simulink model "halfWaveUncontrolledRectifier_RLload"  (R2024b)
settings: Solver=ode23t  StartTime=0.0  StopTime=0.16  MaxStep=1e-4  RelTol=1e-3
libraries: spsVoltageMeasurementLib x3, spsSeriesRLCBranchLib x2, spsACVoltageSourceLib x1, spsDiodeLib x1, spsCurrentMeasurementLib x1, sps_lib x1
settings Model: Creator=farha  LastModifiedBy=farha

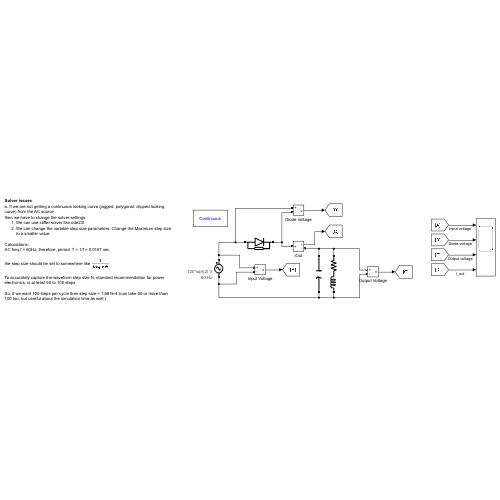
[thumbnail: Simulink's stored preview of the top-level diagram]
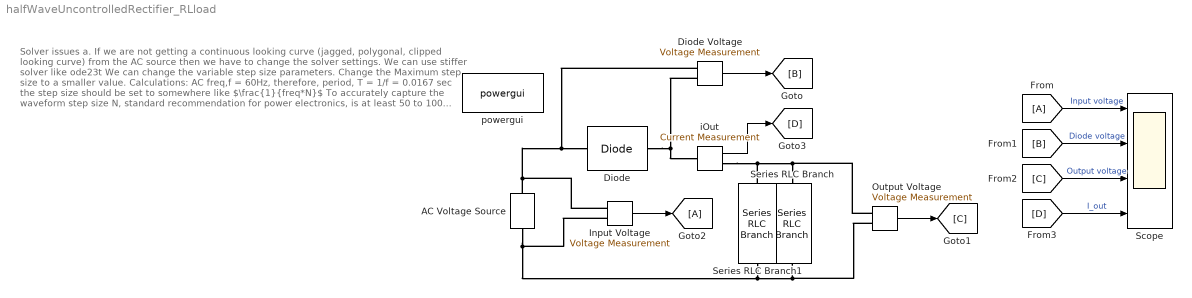
== system halfWaveUncontrolledRectifier_RLload ==
  note: Solver issues
      | a. If we are not getting a continuous looking curve (jagged, polygonal, clipped looking curve) from the AC source
      | then we have to change the solver settings.
      | We can use stiffer solver like ode23t
      | We can change the variable step size parameters. Change the Maximum step size to a smaller value.
      |
      | Calculations:
      | AC freq,f = 60Hz, therefore, period, T = 1/f = 0.0167 sec
      |
      | the step size should be set to somewhere like $\frac{1}{freq*N}$
      |
      | To accurately capture the waveform step size N, standard recommendation for power electronics, is at least 50 to 100 steps
      |
      | So, if we want 100 steps per cycle then step size = 1.667e-4 (can take 50 or more than 100 too, but careful about the simulation time as well.)
  AC Voltage Source : spsACVoltageSourceLib/AC Voltage Source  Amplitude=120*sqrt(2)  Phase=0  Frequency=60  SampleTime=0  Measurements=None  BusType=swing  Pref=10e3  Qref=0  Qmin=-inf  Qmax=+inf
      settings: AttributesFormatString=|
      | %<Amplitude> V
      | %<Frequency> Hz
  Diode : spsDiodeLib/Diode  Ron=0.001  Lon=0  Vf=0.8  IC=0  UseSnubber=0  Rs=500  Cs=250e-9  Measurements=off
  Diode Voltage : spsVoltageMeasurementLib/Voltage Measurement  PhasorSimulation=off  OutputType=Complex  PSBequivalent=0
  From : From
  Goto2 : Goto
  Input Voltage : spsVoltageMeasurementLib/Voltage Measurement  PhasorSimulation=off  OutputType=Complex  PSBequivalent=0
  Output Voltage : spsVoltageMeasurementLib/Voltage Measurement  PhasorSimulation=off  OutputType=Complex  PSBequivalent=0
  Scope : Scope  NumInputPorts=4
  Series RLC Branch : spsSeriesRLCBranchLib/Series RLC Branch  LConnTagsString=__new0  RConnTagsString=__new0  BranchType=RL  Resistance=100  Inductance=0.1  SetiL0=off  InitialCurrent=0  Capacitance=1e-6  Setx0=off  InitialVoltage=0  Measurements=None
  Series RLC Branch1 : spsSeriesRLCBranchLib/Series RLC Branch  LConnTagsString=__new0  RConnTagsString=__new0  BranchType=C  Resistance=5  Inductance=1e-3  SetiL0=off  InitialCurrent=0  Capacitance=220e-6  Setx0=off  InitialVoltage=0  Measurements=None
  iOut : spsCurrentMeasurementLib/Current Measurement  PhasorSimulation=off  OutputType=Complex  PSBequivalent=0
  powergui : sps_lib/powergui  Priority=1  SimulationMode=Continuous  SampleTime=50e-6  frequency=60  Iterations=50  frequencyindice=60  Pbase=100e6  ErrMax=1e-4  UnitsV=kV  UnitsW=MW  buscounter=0  FunctionMessages=off  echomessages=off  EnableUseOfTLC=off  CurrentSourceSwitches=off  DisableSnubberDevices=off  DisableRonSwitches=off  DisableVfSwitches=off  DisplayEquations=off  AutomaticDiscreteSolvers=off  SolverType=Tustin/Backward Euler (TBE)  Interpol=off  ExternalGateDelay=off  methode=off  Ts=100  x0status=blocks  SPID=on  SwTol=0  HookPort=off  NonlinearTolerance=1e-4  nMaxIteration=100  ContinueOnMaxIteration=off  RestoreLinks=warning  ResistiveCurrentMeasurement=off  Frange=[0:2:500]  Ylog=off  Xlog=on  ShowGrid=off  save=off  variable=ZData  structure=0  ZoomFFT=off  StartTime=0.0  cycles=1  DisplayStyle=1  fundamental=60  FreqAxis=off  MaxFrequency=1000  frequencyindicesteady=1  RmsSteady=1  display=off
  wires:
  Diode Voltage/1 -> [B]
  Output Voltage/1 -> [C]
  Input Voltage/1 -> Goto2/1
  iOut/1 -> [D]
  [B] -> Scope/2  "Diode voltage"
  [C] -> Scope/3  "Output voltage"
  [D] -> Scope/4  "I_out"
  From/1 -> Scope/1  "Input voltage"
  connections:
  AC Voltage Source/RConn1 -- Input Voltage/LConn1 -- Diode Voltage/LConn1 -- Diode/LConn1
  Diode/RConn1 -- iOut/LConn1 -- Diode Voltage/LConn2
  iOut/RConn1 -- Series RLC Branch1/LConn1 -- Output Voltage/LConn1 -- Series RLC Branch/LConn1
  AC Voltage Source/LConn1 -- Input Voltage/LConn2 -- Series RLC Branch1/RConn1 -- Output Voltage/LConn2 -- Series RLC Branch/RConn1
